simulink model "MIMO_Alamouti_21_Step1"  (R2026a)
settings: Solver=FixedStepDiscrete  StopTime=inf
PreLoadFcn:
  | EbNo = 5;
  | maxNumErrs = 100;
  | maxNumBits = 1e5;
  | basebandRate=62.5e3;
undefined symbols (not defined in the file): doppler
libraries: commchan3 x3, commmimo x2, commdigbbndpm3 x2, commrandsrc3 x1, commsink2 x1
settings Model: LastModifiedBy=hcha7553
settings DataIOCC: SignalLoggingSaveFormat=ModelDataLogs
settings DebuggingCC: UnderspecifiedInitializationDetection=Classic
settings HardwareCC: ProdHWDeviceType=32-bit Generic
settings GRTTargetCC: CombineOutputUpdateFcns=off  GRTInterface=on

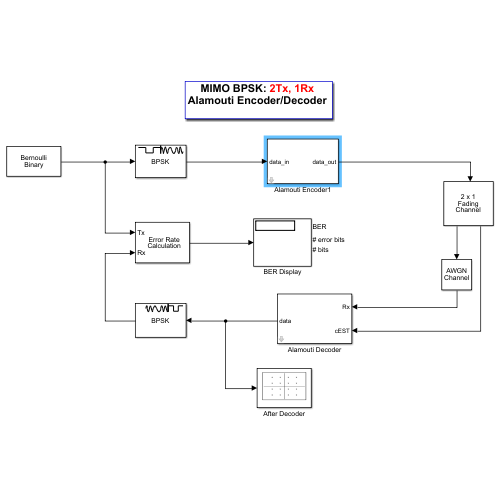
[thumbnail: Simulink's stored preview of the top-level diagram]
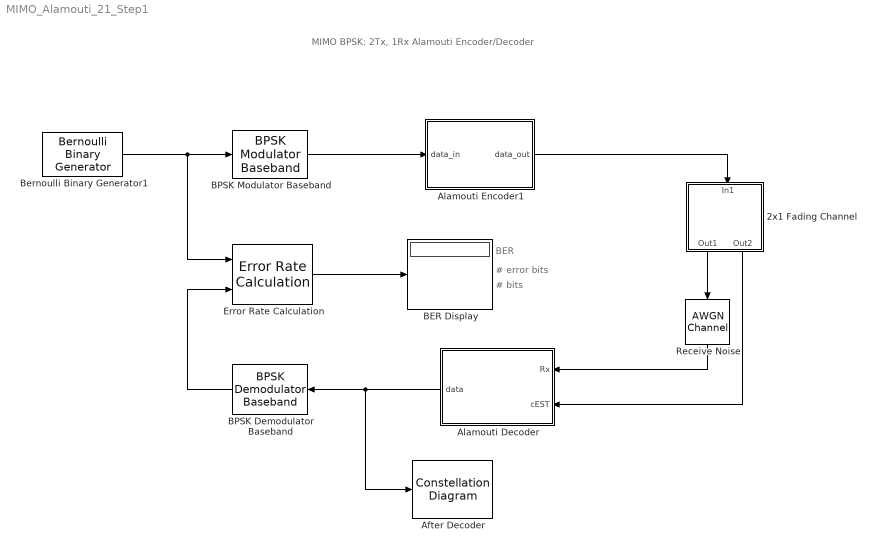
== system MIMO_Alamouti_21_Step1 ==
  note: BER
  note: # error bits
  note: # bits
  note: MIMO BPSK: 2Tx, 1Rx
      | Alamouti Encoder/Decoder
  2x1 Fading Channel : Subsystem
      mask Display: disp('2 x 1\nFading\nChannel');
  After Decoder : ConstellationDiagram  Tag=ScatterPlot  WindowPosition=[258.000000,284.000000,600.000000,600.000000,]  ScopeFrameLocation=window  SamplesPerSymbol=2  SymbolsToDisplaySource=Property  SymbolsToDisplay=1000  ReferenceConstellation=BPSK  Title=After Space time coding  XLimits=[-2.4757 2.6231]  YLimits=[-2.4757 2.6231]  AxesLimits=[-2.4757 2.6231]  DefaultConfigurationName=comm.scopes.ConstellationDiagramBlockCfg
  Alamouti Decoder : Subsystem  mask(Constant){Select_2=2}
      mask prompts: Select_2 "Decoder Selection"
      mask help:
      | Decoder Selection Parameter
      | 1 Simulink Block
      | 2 User Defined Function
  Alamouti Encoder1 : Subsystem  mask(Constant){Select_1=2}
      mask prompts: Select_1 "Encoder Selection"
      mask help:
      | Encoder Selection Parameter:
      | 1 Simulink Block
      | 2 User Defined Function
      mask init:
      | Select=1
  BER Display : Display
  BPSK Demodulator Baseband : commdigbbndpm3/BPSK Demodulator Baseband  DecType=Hard decision  VarSource=Dialog  Variance=1  Ph=0  outDtype=boolean  derotateFactorWordLen=16  derotateFactorDataTypeStr=Inherit: Same word length as input  derotateFactorLastDataTypeStr=Inherit: Same word length as input
  BPSK Modulator Baseband : commdigbbndpm3/BPSK Modulator Baseband  Ph=0  outDtype=double  outWordLen=16  outUDDataType=sfix(16)  outFracLenMode=Best precision  outFracLen=15  outDataTypeStr=double  outLastDataTypeStr=double
  Bernoulli Binary Generator1 : commrandsrc3/Bernoulli Binary Generator  ProbabilityOfZero=.5  SeedSource=Parameter  Seed=61  SampleTime=1/basebandRate  SamplesPerFrame=560  OutputDataType=boolean  SimulateUsing=Interpreted execution
  Error Rate Calculation : commsink2/Error Rate Calculation  N=0  st_delay=0  cp_mode=Entire frame  subframe=[]  PMode=Port  WsName=ErrorVec  RsMode2=off  stop=on  numErr=maxNumErrs  maxBits=maxNumBits
  Receive Noise : commchan3/AWGN Channel  LegacyMode=on  NoiseMethod="Signal to noise ratio  (SNR)"  noiseMode="Signal to noise ratio  (Eb/No)"  EbNo=EbNo  EsNo=5  SNR=EbNo - 10*log10(3)  BitsPerSymbol=1  SignalPower=2  SpecifySymbolPeriod=off  SamplesPerSymbol=1  SymbolPeriod=1/basebandRate  VarianceSource=Parameter  Variance=1  RandomStream=Global stream  Seed=188  SimulateUsing=Code generation
  wires:
  Bernoulli Binary Generator1/1 -> Error Rate Calculation/1, BPSK Modulator Baseband/1
  BPSK Demodulator Baseband/1 -> Error Rate Calculation/2
  Error Rate Calculation/1 -> BER Display/1
  2x1 Fading Channel/1(Out1) -> Receive Noise/1
  BPSK Modulator Baseband/1 -> Alamouti Encoder1/1(data_in)
  Alamouti Encoder1/1(data_out) -> 2x1 Fading Channel/1(In1)
  Receive Noise/1 -> Alamouti Decoder/1(Rx)
  2x1 Fading Channel/2(Out2) -> Alamouti Decoder/2(cEST)
  Alamouti Decoder/1(data) -> BPSK Demodulator Baseband/1, After Decoder/1

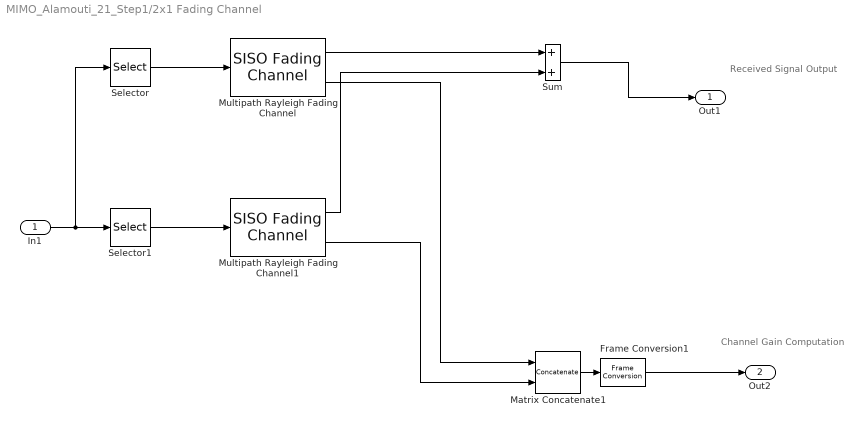
== system MIMO_Alamouti_21_Step1/2x1 Fading Channel ==
  note: Received Signal Output
  note: Channel Gain Computation
  In1 : Inport
  Frame Conversion1 : FrameConversion  OutFrame=Sample-based
  Matrix Concatenate1 : Concatenate  Mode=Multidimensional array  ConcatenateDimension=2
  Multipath Rayleigh Fading Channel : commchan3/SISO Fading Channel  InheritSampleRate=on  SampleRate=1  PathDelays=0  AveragePathGains=0  NormalizePathGains=on  FadingDistribution=Rayleigh  KFactor=3  DirectPathDopplerShift=0  DirectPathInitialPhase=0  MaximumDopplerShift=3  DopplerSpectrum=doppler('Jakes')  RandomStream=mt19937ar with seed  Seed=12345  PathGainsOutputPort=on  ChannelFilterDelayOutputPort=off  SimulateUsing=Interpreted execution  Visualization=Off  PathsForDopplerDisplay=1  SamplesToDisplay=25%
  Multipath Rayleigh Fading Channel1 : commchan3/SISO Fading Channel  InheritSampleRate=on  SampleRate=1  PathDelays=0  AveragePathGains=0  NormalizePathGains=on  FadingDistribution=Rayleigh  KFactor=3  DirectPathDopplerShift=0  DirectPathInitialPhase=0  MaximumDopplerShift=3  DopplerSpectrum=doppler('Jakes')  RandomStream=mt19937ar with seed  Seed=24680  PathGainsOutputPort=on  ChannelFilterDelayOutputPort=off  SimulateUsing=Interpreted execution  Visualization=Off  PathsForDopplerDisplay=1  SamplesToDisplay=25%
  Selector : Selector  NumberOfDimensions=2  InputPortWidth=3  IndexOptions=Select all,Index vector (dialog)  Indices=-1,1  OutputSizes=1
  Selector1 : Selector  NumberOfDimensions=2  InputPortWidth=3  IndexOptions=Select all,Index vector (dialog)  Indices=-1,2  OutputSizes=1
  Sum : Sum
  Out1 : Outport  VectorParamsAs1DForOutWhenUnconnected=off
  Out2 : Outport  Port=2  VectorParamsAs1DForOutWhenUnconnected=off
  wires:
  In1/1 -> Selector1/1, Selector/1
  Multipath Rayleigh Fading Channel1/1 -> Sum/2
  Multipath Rayleigh Fading Channel/1 -> Sum/1
  Multipath Rayleigh Fading Channel1/2 -> Matrix Concatenate1/2
  Multipath Rayleigh Fading Channel/2 -> Matrix Concatenate1/1
  Selector1/1 -> Multipath Rayleigh Fading Channel1/1
  Selector/1 -> Multipath Rayleigh Fading Channel/1
  Sum/1 -> Out1/1
  Matrix Concatenate1/1 -> Frame Conversion1/1
  Frame Conversion1/1 -> Out2/1

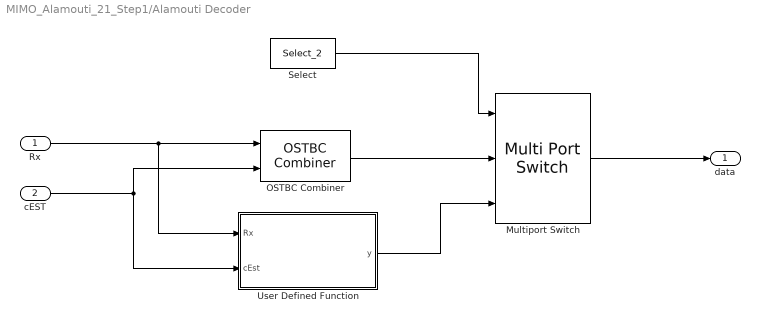
== system MIMO_Alamouti_21_Step1/Alamouti Decoder ==
  Rx : Inport
  cEST : Inport  Port=2
  Multiport Switch : MultiPortSwitch  Inputs=2  SaturateOnIntegerOverflow=off  InputSameDT=off
  OSTBC Combiner : commmimo/OSTBC Combiner  numTx=2  rate=3/4  numRx=1  roundingMode=Floor  overflowMode=Wrap  OvFlMode=off  OvFlModeLastStrValue=off  crossProductWordLen=32  crossProductFracLen=16  crossSumWordLen=32  crossSumFracLen=16  egyProductWordLen=32  egyProductFracLen=16  egySumWordLen=32  egySumFracLen=16  divisionWordLen=32  divisionFracLen=16  divisionDataTypeStr=Inherit: Same as accumulator  divisionLastDataTypeStr=Inherit: Same as accumulator
  Select : Constant  Value=Select_2  VectorParams1D=off  OutMin=1  OutMax=5  OutDataTypeStr=Inherit: Inherit via back propagation
  "User Defined Function " : MATLAB Function  TreatAsAtomicUnit=on
  data : Outport  VectorParamsAs1DForOutWhenUnconnected=off
  wires:
  Select/1 -> Multiport Switch/1
  Rx/1 -> OSTBC Combiner/1, "User Defined Function "/1(Rx)
  cEST/1 -> OSTBC Combiner/2, "User Defined Function "/2(cEst)
  OSTBC Combiner/1 -> Multiport Switch/2
  "User Defined Function "/1(y) -> Multiport Switch/3
  Multiport Switch/1 -> data/1

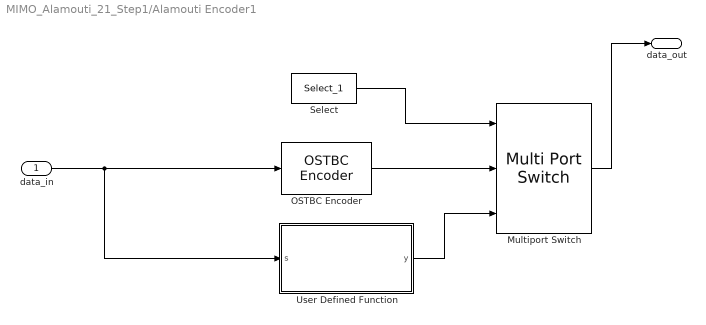
== system MIMO_Alamouti_21_Step1/Alamouti Encoder1 ==
  data_in : Inport
  Multiport Switch : MultiPortSwitch  Inputs=2  SaturateOnIntegerOverflow=off  InputSameDT=off
  OSTBC Encoder : commmimo/OSTBC Encoder  numTx=2  rate=3/4  overflowMode=Wrap  OvFlMode=off  OvFlModeLastStrValue=off
  Select : Constant  Value=Select_1  VectorParams1D=off  OutMin=1  OutMax=5  OutDataTypeStr=Inherit: Inherit via back propagation
  "User Defined Function " : MATLAB Function  TreatAsAtomicUnit=on
  data_out : Outport  VectorParamsAs1DForOutWhenUnconnected=off
  wires:
  data_in/1 -> "User Defined Function "/1(s), OSTBC Encoder/1
  Select/1 -> Multiport Switch/1
  OSTBC Encoder/1 -> Multiport Switch/2
  "User Defined Function "/1(y) -> Multiport Switch/3
  Multiport Switch/1 -> data_out/1

== matlab function MIMO_Alamouti_21_Step1/Alamouti Encoder1/User Defined Function  ==
  data: s input; y output size=[560, 2]
function y = Alamouti_encoder(s) 
%user defined function
y=complex(zeros(560,2));%incomplete code, define output size

== matlab function MIMO_Alamouti_21_Step1/Alamouti Decoder/User Defined Function  ==
  data: Rx input; y output size=[560, 1]; cEst input
function y = Alamouti_decoder(Rx, cEst)
%user defined function
y=complex(zeros(560,1));%imcomplete code
